simulink model "L2_variant9"  (R2026b)
settings: Solver=VariableStepAuto
settings Model: Creator=anna  LastModifiedBy=anna

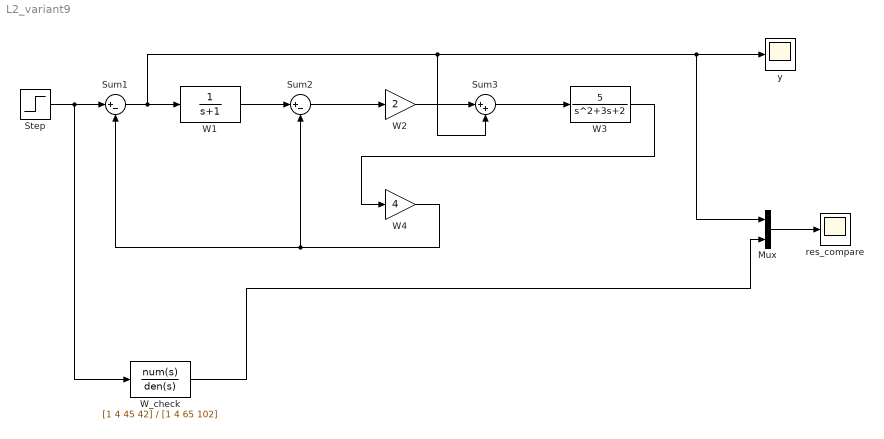
== system L2_variant9 ==
  Mux : Mux  Inputs=2
  Step : Step  Time=0  SampleTime=0
  Sum1 : Sum  Inputs=|+-
  Sum2 : Sum  Inputs=|+-
  Sum3 : Sum  Inputs=|++
  W1 : TransferFcn  Denominator=[1 1]
  W2 : Gain  Gain=2
  W3 : TransferFcn  Numerator=[5]  Denominator=[1 3 2]
  W4 : Gain  Gain=4
  W_check : TransferFcn  Numerator=[1 4 45 42]  Denominator=[1 4 65 102]
  res_compare : Scope
      settings: ActiveDisplayYMinimum=0.27091840711773996  ActiveDisplayYMaximum=1.0810090658758067
  y : Scope
      settings: ActiveDisplayYMinimum=0.25393011787238751  ActiveDisplayYMaximum=1.0828966535697346
  wires:
  Sum1/1 -> Sum3/2, Mux/1, y/1, W1/1
  W1/1 -> Sum2/1
  Sum2/1 -> W2/1
  Step/1 -> W_check/1, Sum1/1
  W4/1 -> Sum2/2, Sum1/2
  W3/1 -> W4/1
  Sum3/1 -> W3/1
  W2/1 -> Sum3/1
  W_check/1 -> Mux/2
  Mux/1 -> res_compare/1
